simulink library "loco_native_lib"  (R2024b)
settings: Solver=VariableStepAuto  StartTime=0.0  StopTime=10.0  RelTol=1e-3
undefined symbols (not defined in the file): P, PN
libraries: fl_lib x96, nesl_utility x44, $bdroot x21, simulink x2, sdl_lib x1, batteryecm_lib x1
(part 2 of 2)

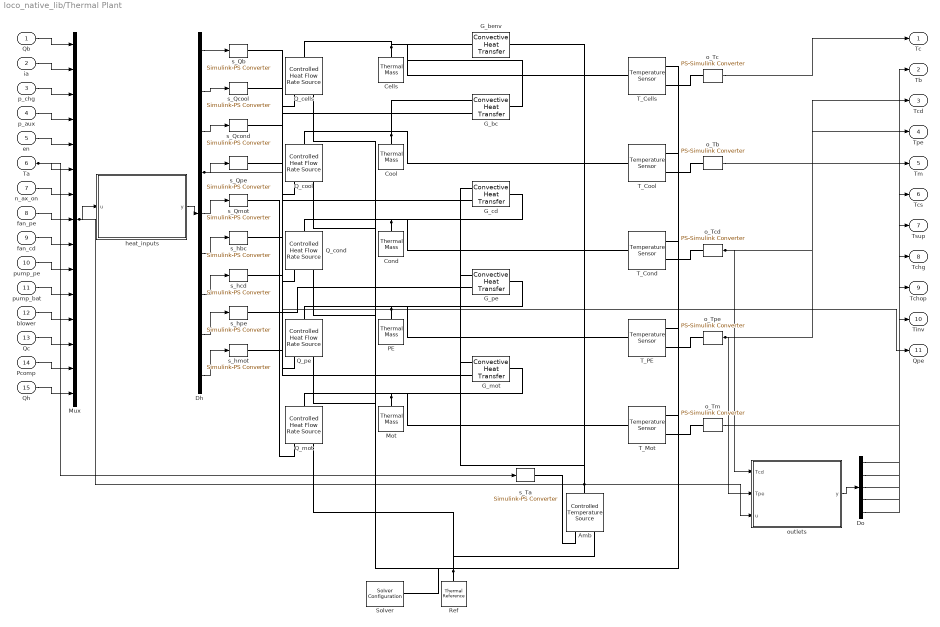
== system loco_native_lib/Thermal Plant ==
  Qb : Inport
  ia : Inport  Port=2
  p_chg : Inport  Port=3
  p_aux : Inport  Port=4
  en : Inport  Port=5
  Ta : Inport  Port=6
  n_ax_on : Inport  Port=7
  fan_pe : Inport  Port=8
  fan_cd : Inport  Port=9
  pump_pe : Inport  Port=10
  pump_bat : Inport  Port=11
  blower : Inport  Port=12
  Qc : Inport  Port=13
  Pcomp : Inport  Port=14
  Qh : Inport  Port=15
  Amb : fl_lib/Thermal/Thermal Sources/Controlled Temperature Source
  Cells : fl_lib/Thermal/Thermal Elements/Thermal Mass  mass_type=foundation.enum.constant_variable.constant  mass=TH.C_bat kg  sp_heat=1 J/(K*kg)  mass_min=1e-6 kg  num_ports=foundation.enum.numPorts2.one  m_specify=off  m_priority=High  m=1 kg  m_nominal_specify=off  m_nominal_value=1  m_nominal_unit=kg  T_specify=on  T_priority=High  T=TH.T0_bat K  T_nominal_specify=off  T_nominal_value=1  T_nominal_unit=K  Q_specify=off  Q_priority=None  Q=0 W  Q_nominal_specify=off  Q_nominal_value=1  Q_nominal_unit=W
  Cond : fl_lib/Thermal/Thermal Elements/Thermal Mass  mass_type=foundation.enum.constant_variable.constant  mass=TH.C_cd kg  sp_heat=1 J/(K*kg)  mass_min=1e-6 kg  num_ports=foundation.enum.numPorts2.one  m_specify=off  m_priority=High  m=1 kg  m_nominal_specify=off  m_nominal_value=1  m_nominal_unit=kg  T_specify=on  T_priority=High  T=TH.T_amb K  T_nominal_specify=off  T_nominal_value=1  T_nominal_unit=K  Q_specify=off  Q_priority=None  Q=0 W  Q_nominal_specify=off  Q_nominal_value=1  Q_nominal_unit=W
  Cool : fl_lib/Thermal/Thermal Elements/Thermal Mass  mass_type=foundation.enum.constant_variable.constant  mass=TH.C_bc kg  sp_heat=1 J/(K*kg)  mass_min=1e-6 kg  num_ports=foundation.enum.numPorts2.one  m_specify=off  m_priority=High  m=1 kg  m_nominal_specify=off  m_nominal_value=1  m_nominal_unit=kg  T_specify=on  T_priority=High  T=TH.T0_bat K  T_nominal_specify=off  T_nominal_value=1  T_nominal_unit=K  Q_specify=off  Q_priority=None  Q=0 W  Q_nominal_specify=off  Q_nominal_value=1  Q_nominal_unit=W
  Dh : Demux  Outputs=9
  Do : Demux  Outputs=5
  G_bc : fl_lib/Thermal/Thermal Elements/Convective Heat Transfer  thermal_type=foundation.enum.constant_variable.variable  area=1 m^2  heat_tr_coeff=20 W/(K*m^2)  min_heat_tr_coeff=1e-3 W/(K*m^2)  T_specify=off  T_priority=None  T=0 K  T_nominal_specify=off  T_nominal_value=1  T_nominal_unit=K  Q_specify=off  Q_priority=None  Q=0 W  Q_nominal_specify=off  Q_nominal_value=1  Q_nominal_unit=W
      settings: InternalSimscapePortConfiguration="{\"Bottom\":[],\"Left\":[{\"id\":\"A\",\"label\":\"A\",\"type\":\"foundation.thermal.thermal\"},{\"id\":\"var_heat_tr_coeff\",\"label\":\"K\",\"type\":\"input\"}],\"Right\":[{\"id\":\"B\",\"label\":\"B\",\"type\":\"foundation.thermal.thermal\"}],\"Top\":[]}"
  G_benv : fl_lib/Thermal/Thermal Elements/Convective Heat Transfer  thermal_type=foundation.enum.constant_variable.constant  area=1 m^2  heat_tr_coeff=TH.UA_benv W/(K*m^2)  min_heat_tr_coeff=1e-3 W/(K*m^2)  T_specify=off  T_priority=None  T=0 K  T_nominal_specify=off  T_nominal_value=1  T_nominal_unit=K  Q_specify=off  Q_priority=None  Q=0 W  Q_nominal_specify=off  Q_nominal_value=1  Q_nominal_unit=W
  G_cd : fl_lib/Thermal/Thermal Elements/Convective Heat Transfer  thermal_type=foundation.enum.constant_variable.variable  area=1 m^2  heat_tr_coeff=20 W/(K*m^2)  min_heat_tr_coeff=1e-3 W/(K*m^2)  T_specify=off  T_priority=None  T=0 K  T_nominal_specify=off  T_nominal_value=1  T_nominal_unit=K  Q_specify=off  Q_priority=None  Q=0 W  Q_nominal_specify=off  Q_nominal_value=1  Q_nominal_unit=W
      settings: InternalSimscapePortConfiguration="{\"Bottom\":[],\"Left\":[{\"id\":\"A\",\"label\":\"A\",\"type\":\"foundation.thermal.thermal\"},{\"id\":\"var_heat_tr_coeff\",\"label\":\"K\",\"type\":\"input\"}],\"Right\":[{\"id\":\"B\",\"label\":\"B\",\"type\":\"foundation.thermal.thermal\"}],\"Top\":[]}"
  G_mot : fl_lib/Thermal/Thermal Elements/Convective Heat Transfer  thermal_type=foundation.enum.constant_variable.variable  area=1 m^2  heat_tr_coeff=20 W/(K*m^2)  min_heat_tr_coeff=1e-3 W/(K*m^2)  T_specify=off  T_priority=None  T=0 K  T_nominal_specify=off  T_nominal_value=1  T_nominal_unit=K  Q_specify=off  Q_priority=None  Q=0 W  Q_nominal_specify=off  Q_nominal_value=1  Q_nominal_unit=W
      settings: InternalSimscapePortConfiguration="{\"Bottom\":[],\"Left\":[{\"id\":\"A\",\"label\":\"A\",\"type\":\"foundation.thermal.thermal\"},{\"id\":\"var_heat_tr_coeff\",\"label\":\"K\",\"type\":\"input\"}],\"Right\":[{\"id\":\"B\",\"label\":\"B\",\"type\":\"foundation.thermal.thermal\"}],\"Top\":[]}"
  G_pe : fl_lib/Thermal/Thermal Elements/Convective Heat Transfer  thermal_type=foundation.enum.constant_variable.variable  area=1 m^2  heat_tr_coeff=20 W/(K*m^2)  min_heat_tr_coeff=1e-3 W/(K*m^2)  T_specify=off  T_priority=None  T=0 K  T_nominal_specify=off  T_nominal_value=1  T_nominal_unit=K  Q_specify=off  Q_priority=None  Q=0 W  Q_nominal_specify=off  Q_nominal_value=1  Q_nominal_unit=W
      settings: InternalSimscapePortConfiguration="{\"Bottom\":[],\"Left\":[{\"id\":\"A\",\"label\":\"A\",\"type\":\"foundation.thermal.thermal\"},{\"id\":\"var_heat_tr_coeff\",\"label\":\"K\",\"type\":\"input\"}],\"Right\":[{\"id\":\"B\",\"label\":\"B\",\"type\":\"foundation.thermal.thermal\"}],\"Top\":[]}"
  Mot : fl_lib/Thermal/Thermal Elements/Thermal Mass  mass_type=foundation.enum.constant_variable.constant  mass=TH.C_mot kg  sp_heat=1 J/(K*kg)  mass_min=1e-6 kg  num_ports=foundation.enum.numPorts2.one  m_specify=off  m_priority=High  m=1 kg  m_nominal_specify=off  m_nominal_value=1  m_nominal_unit=kg  T_specify=on  T_priority=High  T=TH.T_amb K  T_nominal_specify=off  T_nominal_value=1  T_nominal_unit=K  Q_specify=off  Q_priority=None  Q=0 W  Q_nominal_specify=off  Q_nominal_value=1  Q_nominal_unit=W
  Mux : Mux  Inputs=15
  PE : fl_lib/Thermal/Thermal Elements/Thermal Mass  mass_type=foundation.enum.constant_variable.constant  mass=TH.C_pe kg  sp_heat=1 J/(K*kg)  mass_min=1e-6 kg  num_ports=foundation.enum.numPorts2.one  m_specify=off  m_priority=High  m=1 kg  m_nominal_specify=off  m_nominal_value=1  m_nominal_unit=kg  T_specify=on  T_priority=High  T=TH.T_amb K  T_nominal_specify=off  T_nominal_value=1  T_nominal_unit=K  Q_specify=off  Q_priority=None  Q=0 W  Q_nominal_specify=off  Q_nominal_value=1  Q_nominal_unit=W
  Q_cells : fl_lib/Thermal/Thermal Sources/Controlled Heat Flow Rate Source
  Q_cond : fl_lib/Thermal/Thermal Sources/Controlled Heat Flow Rate Source
  Q_cool : fl_lib/Thermal/Thermal Sources/Controlled Heat Flow Rate Source
  Q_mot : fl_lib/Thermal/Thermal Sources/Controlled Heat Flow Rate Source
  Q_pe : fl_lib/Thermal/Thermal Sources/Controlled Heat Flow Rate Source
  Ref : fl_lib/Thermal/Thermal Elements/Thermal Reference
  Solver : nesl_utility/Solver Configuration  PhysicalDomain=network_engine_domain  SubClassName=solver  LeftPortType=input  RightPortType=generic  Tones=[]  Harmonics=[]  SimulateNoise=off  Profile=off  UseLocalSampling=off  EnableSwitchedLinearOptims=on  FrequencyDomain=off  UseCCode=off  RelTol=0.001  AbsTol=0.001  MinStep=1e-09  ToWorkspace=off  RevertToSquareIcSolve=off  NumHomotopyIterations=100  PhasorMode=off  PhasorModeNumHarmonics=1  ConsistencySolver=NEWTON_XTOL_AFTER_FTOL  IndexReductionMethod=DerivativeReplacement  DoDC=off  ResidualTolerance=1e-09  ConsistencyTolSource=GLOBAL  ConsistencyAbsTol=0.001  ConsistencyRelTol=0.001  ConsistencyTolFactor=0.001  UseLocalSolver=off  LocalSolverChoice=NE_BACKWARD_EULER_ADVANCER  ResolveIndetEquations=on  FunctionEvalNumThread=1  LocalSolverSampleTime=0.001  DoFixedCost=off  MaxNonlinIter=3  MaxModeIter=2  ComputeImpulses=off  ImpulseIterations=2  LinearAlgebra=auto  LinearAlgebraNumThread=0  EquationFormulation=NE_TIME_EF  DelaysMemoryBudget=1024  AutomaticFiltering=on  FilteringTimeConstant=0.001  PartitionStorageMethod=AS_NEEDED  PartitionMemoryBudget=1024  PartitionMethod=ROBUST  MultibodyUseLocalSolver=off  MultibodyLocalSolverChoice=ODE1  MultibodyLocalSolverSampleTime=0.001
  T_Cells : fl_lib/Thermal/Thermal Sensors/Temperature Sensor  temperature_measure=foundation.enum.MeasurementReference.difference
  T_Cond : fl_lib/Thermal/Thermal Sensors/Temperature Sensor  temperature_measure=foundation.enum.MeasurementReference.difference
  T_Cool : fl_lib/Thermal/Thermal Sensors/Temperature Sensor  temperature_measure=foundation.enum.MeasurementReference.difference
  T_Mot : fl_lib/Thermal/Thermal Sensors/Temperature Sensor  temperature_measure=foundation.enum.MeasurementReference.difference
  T_PE : fl_lib/Thermal/Thermal Sensors/Temperature Sensor  temperature_measure=foundation.enum.MeasurementReference.difference
  heat_inputs : MATLAB Function  TreatAsAtomicUnit=on
  o_Tb : nesl_utility/PS-Simulink Converter  PhysicalDomain=network_engine_domain  SubClassName=ps_output  LeftPortType=input  RightPortType=output  PseudoPeriodic=off  Frequencies=[]  VectorFormat=inherit  Unit=K  AffineConversion=off
  o_Tc : nesl_utility/PS-Simulink Converter  PhysicalDomain=network_engine_domain  SubClassName=ps_output  LeftPortType=input  RightPortType=output  PseudoPeriodic=off  Frequencies=[]  VectorFormat=inherit  Unit=K  AffineConversion=off
  o_Tcd : nesl_utility/PS-Simulink Converter  PhysicalDomain=network_engine_domain  SubClassName=ps_output  LeftPortType=input  RightPortType=output  PseudoPeriodic=off  Frequencies=[]  VectorFormat=inherit  Unit=K  AffineConversion=off
  o_Tm : nesl_utility/PS-Simulink Converter  PhysicalDomain=network_engine_domain  SubClassName=ps_output  LeftPortType=input  RightPortType=output  PseudoPeriodic=off  Frequencies=[]  VectorFormat=inherit  Unit=K  AffineConversion=off
  o_Tpe : nesl_utility/PS-Simulink Converter  PhysicalDomain=network_engine_domain  SubClassName=ps_output  LeftPortType=input  RightPortType=output  PseudoPeriodic=off  Frequencies=[]  VectorFormat=inherit  Unit=K  AffineConversion=off
  outlets : MATLAB Function  TreatAsAtomicUnit=on
  s_Qb : nesl_utility/Simulink-PS Converter  PhysicalDomain=network_engine_domain  SubClassName=ps_input  LeftPortType=input  RightPortType=output  PseudoPeriodic=off  Frequencies=[]  NoiseDistribution=none  NoiseParameters=[]  Unit=W  AffineConversion=off  FilteringAndDerivatives=provide  SimscapeFilterOrder=1  InputFilterTimeConstant=0.001  UdotUserProvided=0
  s_Qcond : nesl_utility/Simulink-PS Converter  PhysicalDomain=network_engine_domain  SubClassName=ps_input  LeftPortType=input  RightPortType=output  PseudoPeriodic=off  Frequencies=[]  NoiseDistribution=none  NoiseParameters=[]  Unit=W  AffineConversion=off  FilteringAndDerivatives=provide  SimscapeFilterOrder=1  InputFilterTimeConstant=0.001  UdotUserProvided=0
  s_Qcool : nesl_utility/Simulink-PS Converter  PhysicalDomain=network_engine_domain  SubClassName=ps_input  LeftPortType=input  RightPortType=output  PseudoPeriodic=off  Frequencies=[]  NoiseDistribution=none  NoiseParameters=[]  Unit=W  AffineConversion=off  FilteringAndDerivatives=provide  SimscapeFilterOrder=1  InputFilterTimeConstant=0.001  UdotUserProvided=0
  s_Qmot : nesl_utility/Simulink-PS Converter  PhysicalDomain=network_engine_domain  SubClassName=ps_input  LeftPortType=input  RightPortType=output  PseudoPeriodic=off  Frequencies=[]  NoiseDistribution=none  NoiseParameters=[]  Unit=W  AffineConversion=off  FilteringAndDerivatives=provide  SimscapeFilterOrder=1  InputFilterTimeConstant=0.001  UdotUserProvided=0
  s_Qpe : nesl_utility/Simulink-PS Converter  PhysicalDomain=network_engine_domain  SubClassName=ps_input  LeftPortType=input  RightPortType=output  PseudoPeriodic=off  Frequencies=[]  NoiseDistribution=none  NoiseParameters=[]  Unit=W  AffineConversion=off  FilteringAndDerivatives=provide  SimscapeFilterOrder=1  InputFilterTimeConstant=0.001  UdotUserProvided=0
  s_Ta : nesl_utility/Simulink-PS Converter  PhysicalDomain=network_engine_domain  SubClassName=ps_input  LeftPortType=input  RightPortType=output  PseudoPeriodic=off  Frequencies=[]  NoiseDistribution=none  NoiseParameters=[]  Unit=K  AffineConversion=off  FilteringAndDerivatives=provide  SimscapeFilterOrder=1  InputFilterTimeConstant=0.001  UdotUserProvided=0
  s_hbc : nesl_utility/Simulink-PS Converter  PhysicalDomain=network_engine_domain  SubClassName=ps_input  LeftPortType=input  RightPortType=output  PseudoPeriodic=off  Frequencies=[]  NoiseDistribution=none  NoiseParameters=[]  Unit=W/(m^2*K)  AffineConversion=off  FilteringAndDerivatives=provide  SimscapeFilterOrder=1  InputFilterTimeConstant=0.001  UdotUserProvided=0
  s_hcd : nesl_utility/Simulink-PS Converter  PhysicalDomain=network_engine_domain  SubClassName=ps_input  LeftPortType=input  RightPortType=output  PseudoPeriodic=off  Frequencies=[]  NoiseDistribution=none  NoiseParameters=[]  Unit=W/(m^2*K)  AffineConversion=off  FilteringAndDerivatives=provide  SimscapeFilterOrder=1  InputFilterTimeConstant=0.001  UdotUserProvided=0
  s_hmot : nesl_utility/Simulink-PS Converter  PhysicalDomain=network_engine_domain  SubClassName=ps_input  LeftPortType=input  RightPortType=output  PseudoPeriodic=off  Frequencies=[]  NoiseDistribution=none  NoiseParameters=[]  Unit=W/(m^2*K)  AffineConversion=off  FilteringAndDerivatives=provide  SimscapeFilterOrder=1  InputFilterTimeConstant=0.001  UdotUserProvided=0
  s_hpe : nesl_utility/Simulink-PS Converter  PhysicalDomain=network_engine_domain  SubClassName=ps_input  LeftPortType=input  RightPortType=output  PseudoPeriodic=off  Frequencies=[]  NoiseDistribution=none  NoiseParameters=[]  Unit=W/(m^2*K)  AffineConversion=off  FilteringAndDerivatives=provide  SimscapeFilterOrder=1  InputFilterTimeConstant=0.001  UdotUserProvided=0
  Tc : Outport
  Tb : Outport  Port=2
  Tcd : Outport  Port=3
  Tpe : Outport  Port=4
  Tm : Outport  Port=5
  Tcs : Outport  Port=6
  Tsup : Outport  Port=7
  Tchg : Outport  Port=8
  Tchop : Outport  Port=9
  Tinv : Outport  Port=10
  Qpe : Outport  Port=11
  wires:
  Qb/1 -> Mux/1
  ia/1 -> Mux/2
  p_chg/1 -> Mux/3
  p_aux/1 -> Mux/4
  en/1 -> Mux/5
  Ta/1 -> Mux/6, s_Ta/1
  n_ax_on/1 -> Mux/7
  fan_pe/1 -> Mux/8
  fan_cd/1 -> Mux/9
  pump_pe/1 -> Mux/10
  pump_bat/1 -> Mux/11
  blower/1 -> Mux/12
  Qc/1 -> Mux/13
  Pcomp/1 -> Mux/14
  Qh/1 -> Mux/15
  Mux/1 -> heat_inputs/1(u), outlets/3(u)
  heat_inputs/1(y) -> Dh/1
  Dh/1 -> s_Qb/1
  Dh/2 -> s_Qcool/1
  Dh/3 -> s_Qcond/1
  Dh/4 -> s_Qpe/1, Qpe/1
  Dh/5 -> s_Qmot/1
  Dh/6 -> s_hbc/1
  Dh/7 -> s_hcd/1
  Dh/8 -> s_hpe/1
  Dh/9 -> s_hmot/1
  o_Tcd/1 -> outlets/1(Tcd), Tcd/1
  o_Tpe/1 -> outlets/2(Tpe), Tpe/1
  outlets/1(y) -> Do/1
  o_Tc/1 -> Tc/1
  o_Tb/1 -> Tb/1
  o_Tm/1 -> Tm/1
  Do/1 -> Tcs/1
  Do/2 -> Tsup/1
  Do/3 -> Tchg/1
  Do/4 -> Tchop/1
  Do/5 -> Tinv/1
  connections:
  Solver/RConn1 -- Amb/RConn2 -- Q_cells/RConn2 -- T_Cells/RConn1 -- Q_cool/RConn2 -- T_Cool/RConn1 -- Q_cond/RConn2 -- T_Cond/RConn1 -- Q_pe/RConn2 -- T_PE/RConn1 -- Q_mot/RConn2 -- Ref/LConn1 -- T_Mot/RConn1
  s_Ta/RConn1 -- Amb/RConn1
  s_Qb/RConn1 -- Q_cells/RConn1
  Q_cells/LConn1 -- T_Cells/LConn1 -- G_benv/LConn1 -- Cells/LConn1 -- G_bc/RConn1
  T_Cells/RConn2 -- o_Tc/LConn1
  s_Qcool/RConn1 -- Q_cool/RConn1
  Q_cool/LConn1 -- T_Cool/LConn1 -- Cool/LConn1 -- G_bc/LConn1
  T_Cool/RConn2 -- o_Tb/LConn1
  s_Qcond/RConn1 -- Q_cond/RConn1
  Q_cond/LConn1 -- T_Cond/LConn1 -- Cond/LConn1 -- G_cd/RConn1
  T_Cond/RConn2 -- o_Tcd/LConn1
  s_Qpe/RConn1 -- Q_pe/RConn1
  Q_pe/LConn1 -- T_PE/LConn1 -- PE/LConn1 -- G_pe/RConn1
  T_PE/RConn2 -- o_Tpe/LConn1
  s_Qmot/RConn1 -- Q_mot/RConn1
  Q_mot/LConn1 -- T_Mot/LConn1 -- Mot/LConn1 -- G_mot/RConn1
  T_Mot/RConn2 -- o_Tm/LConn1
  G_benv/RConn1 -- G_cd/LConn1 -- G_pe/LConn1 -- Amb/LConn1 -- G_mot/LConn1
  s_hbc/RConn1 -- G_bc/LConn2
  s_hcd/RConn1 -- G_cd/LConn2
  s_hpe/RConn1 -- G_pe/LConn2
  s_hmot/RConn1 -- G_mot/LConn2

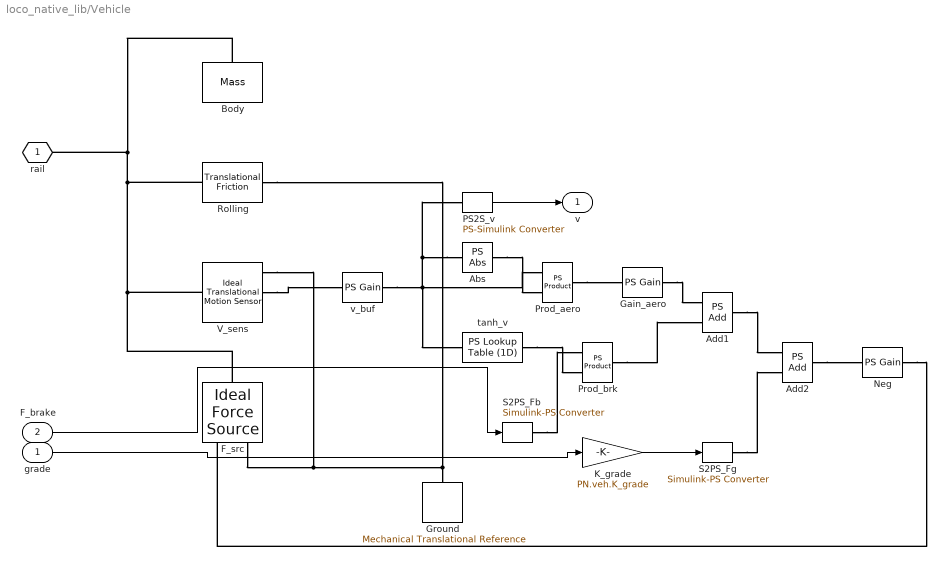
== system loco_native_lib/Vehicle ==
  grade : Inport
  F_brake : Inport  Port=2
  Abs : fl_lib/Physical Signals/Nonlinear Operators/PS Abs
      settings: InternalSimscapePortConfiguration="{\"Bottom\":[],\"Left\":[{\"id\":\"I\",\"label\":\"\",\"type\":\"input\"}],\"Right\":[{\"id\":\"O\",\"label\":\"\",\"type\":\"output\"}],\"Top\":[]}"
  Add1 : fl_lib/Physical Signals/Functions/PS Add
  Add2 : fl_lib/Physical Signals/Functions/PS Add
  Body : fl_lib/Mechanical/Translational Elements/Mass  mass=PN.veh.m_eff kg  num_ports=foundation.enum.numPorts2.one  v_specify=on  v_priority=High  v=PN.veh.v0 m/s  v_nominal_specify=off  v_nominal_value=1  v_nominal_unit=m/s  f_specify=off  f_priority=None  f=0 N  f_nominal_specify=off  f_nominal_value=1  f_nominal_unit=N
  F_src : fl_lib/Mechanical/Mechanical Sources/Ideal Force Source
  Gain_aero : fl_lib/Physical Signals/Functions/PS Gain  gain=PN.veh.k_aero N*s^2/m^2
  Ground : fl_lib/Mechanical/Translational Elements/Mechanical Translational Reference
  K_grade : Gain  Gain=PN.veh.K_grade
  Neg : fl_lib/Physical Signals/Functions/PS Gain  gain=-1
  PS2S_v : nesl_utility/PS-Simulink Converter  PhysicalDomain=network_engine_domain  SubClassName=ps_output  LeftPortType=input  RightPortType=output  PseudoPeriodic=off  Frequencies=[]  VectorFormat=inherit  Unit=m/s  AffineConversion=off
  Prod_aero : fl_lib/Physical Signals/Functions/PS Product
  Prod_brk : fl_lib/Physical Signals/Functions/PS Product
  Rolling : fl_lib/Mechanical/Translational Elements/Translational Friction  brkwy_frc=PN.veh.F_roll N  brkwy_vel=1 m/s  Col_frc=PN.veh.F_roll N  visc_coef=0 N*s/m  v_specify=off  v_priority=None  v=0 m/s  v_nominal_specify=off  v_nominal_value=1  v_nominal_unit=m/s  f_specify=off  f_priority=None  f=0 N  f_nominal_specify=off  f_nominal_value=1  f_nominal_unit=N
      settings: InternalSimscapePortConfiguration="{\"Bottom\":[],\"Left\":[{\"id\":\"R\",\"label\":\"R\",\"type\":\"foundation.mechanical.translational.translational\"}],\"Right\":[{\"id\":\"C\",\"label\":\"C\",\"type\":\"foundation.mechanical.translational.translational\"}],\"Top\":[]}"
  S2PS_Fb : nesl_utility/Simulink-PS Converter  PhysicalDomain=network_engine_domain  SubClassName=ps_input  LeftPortType=input  RightPortType=output  PseudoPeriodic=off  Frequencies=[]  NoiseDistribution=none  NoiseParameters=[]  Unit=N  AffineConversion=off  FilteringAndDerivatives=provide  SimscapeFilterOrder=1  InputFilterTimeConstant=0.001  UdotUserProvided=0
  S2PS_Fg : nesl_utility/Simulink-PS Converter  PhysicalDomain=network_engine_domain  SubClassName=ps_input  LeftPortType=input  RightPortType=output  PseudoPeriodic=off  Frequencies=[]  NoiseDistribution=none  NoiseParameters=[]  Unit=N  AffineConversion=off  FilteringAndDerivatives=provide  SimscapeFilterOrder=1  InputFilterTimeConstant=0.001  UdotUserProvided=0
  V_sens : fl_lib/Mechanical/Mechanical Sensors/Ideal Translational Motion Sensor  reference=foundation.enum.MeasurementReference.difference  acceleration_port=false  velocity_port=true  position_port=true  offset=0 m
  tanh_v : fl_lib/Physical Signals/Lookup Tables/PS Lookup Table (1D)  x=PN.veh.tanh_x m/s  f=PN.veh.tanh_f  interp_method=simscape.enum.interpolation.linear  extrap_method=simscape.enum.extrapolation.linear
  v_buf : fl_lib/Physical Signals/Functions/PS Gain  gain=1
  rail : PMIOPort  Side=Left
  v : Outport
  wires:
  grade/1 -> K_grade/1
  K_grade/1 -> S2PS_Fg/1
  F_brake/1 -> S2PS_Fb/1
  PS2S_v/1 -> v/1
  connections:
  Abs/LConn1 -- v_buf/RConn1 -- Prod_aero/LConn1 -- tanh_v/LConn1 -- PS2S_v/LConn1
  Abs/RConn1 -- Prod_aero/LConn2
  Prod_aero/RConn1 -- Gain_aero/LConn1
  S2PS_Fb/RConn1 -- Prod_brk/LConn1
  tanh_v/RConn1 -- Prod_brk/LConn2
  Gain_aero/RConn1 -- Add1/LConn1
  Prod_brk/RConn1 -- Add1/LConn2
  Add1/RConn1 -- Add2/LConn1
  S2PS_Fg/RConn1 -- Add2/LConn2
  Add2/RConn1 -- Neg/LConn1
  Body/LConn1 -- F_src/LConn1 -- V_sens/LConn1 -- Rolling/LConn1 -- rail/RConn1
  Rolling/RConn1 -- F_src/RConn2 -- V_sens/RConn1 -- Ground/LConn1
  V_sens/RConn2 -- v_buf/LConn1
  Neg/RConn1 -- F_src/RConn1

== matlab function loco_native_lib/LCC/lcc ==
  data: u input size=[9 1]; y output; L parameter
function y = lcc(u, L)
persistent xi
if isempty(xi), xi = 0; end
v_ref = u(1); v = u(2); Vbat = u(3); k_dis = u(4); k_chg = u(5);
m_trail = u(6); trac = u(7); n_ax_on = u(8); n_str = u(9);
mt = max(m_trail, 0);
m_tot = L.m_loco + mt;
m_eff = L.k_rot_loco*L.m_loco + L.k_rot_trail*mt;
Kp = 2*L.zeta*L.wn*m_eff;
Ki = L.wn^2*m_eff;
nax = min(max(n_ax_on, 0), L.N_ax);
fstr = min(max(n_str, 0), L.N_str_nom)/L.N_str_nom;
TE_adh = L.mu_adh*L.m_loco*L.g*nax/L.N_ax;
e = v_ref - v;
TE_raw = Kp*e + xi;
vabs = max(abs(v), L.v_floor);
P_dis = trac*min(L.P_trac_max*nax/L.N_ax, L.I_dis_max*fstr*k_dis*Vbat*L.eta_drv);
P_reg = min(L.P_trac_max*nax/L.N_ax, L.I_chg_max*fstr*k_chg*Vbat/L.eta_drv);
TE_mot_lim = min(TE_adh, P_dis/vabs);
TE_reg_lim = min(TE_adh, P_reg/vabs)*min(abs(v)/L.v_blend, 1);
TE_cmd = min(max(TE_raw, -TE_adh), TE_mot_lim);
TE_el = max(TE_cmd, -TE_reg_lim);
F_park = L.mu_park*m_tot*L.g;
if v_ref < 0.01
    F_hold = F_park;
    dxi = -xi/1;
else
    F_hold = F_park*min(max(-v/L.v_rb, 0), 1);
    dxi = Ki*e + (TE_cmd - TE_raw)/L.T_aw;
end
xi = xi + L.Ts*dxi;
TE_each = TE_el/max(nax, 1);
y = [TE_each; TE_each*min(max(nax - 3, 0), 1); TE_el - TE_cmd + F_hold];
end

== matlab function loco_native_lib/Chopper FW/fw ==
  data: TE_ref input size=[1 1]; Va output; i_a input size=[1 1]; v input size=[1 1]; Vdc input size=[1 1]; A parameter
function Va = fw(TE_ref, i_a, v, Vdc, A)
wm = A.G*v/A.r_w;
kphi = A.Kphi_sat*(1 - exp(-max(abs(i_a), A.If_min)/A.I0));
E = kphi*wm;
Vmax = min(A.D_max*max(Vdc, 0), A.V_mot_max);
Tm_lim = A.P_ax_max/max(abs(wm), A.w_floor);
Tm_ref = min(max(TE_ref*A.r_w/A.G, -Tm_lim), Tm_lim);
Iref = sign(Tm_ref)*interp1(A.T_tab, A.I_tab, min(abs(Tm_ref), A.T_tab(end)));
Iref = min(max(Iref, -A.I_max), A.I_max);
Va = min(max(E + A.R_m*i_a + A.Kp_i*(Iref - i_a), 0), Vmax);
end

== matlab function loco_native_lib/Charger FW/chg ==
  data: u input size=[5 1]; i output; P_max parameter; I_max parameter; I_bms parameter; soc_max parameter; soc_band parameter; V_floor parameter; N_str_nom parameter
function i = chg(u, P_max, I_max, I_bms, soc_max, soc_band, V_floor, N_str_nom)
P = u(1); k = u(2); soc = u(3); n_str = u(4); V = u(5);
Ilim = min(I_max, I_bms*k*n_str/N_str_nom);
Ip = min(max(P, 0), P_max)/max(V, V_floor);
taper = min(max((soc_max - soc)/soc_band, 0), 1);
i = min(Ip, Ilim)*taper;
end

== matlab function loco_native_lib/Thermal Plant/heat_inputs ==
  data: u input size=[15 1]; y output; TH parameter; f_ram parameter
function y = heat_inputs(u, TH, f_ram)
Qb = u(1); ia = u(2); p_chg = u(3); p_aux = u(4); en = u(5);
n_ax = u(7); fan_pe = u(8); fan_cd = u(9); pump_pe = u(10); pump_bat = u(11);
blower = u(12); Qc = u(13); Pcomp = u(14); Qh = u(15);
Qchop = n_ax*(TH.a_loss*abs(ia) + TH.b_loss*ia^2);
Qchg = max(p_chg, 0)*(1/TH.eta_chg - 1);
Qpe = Qchop + Qchg + TH.k_aux_pe*p_aux + TH.Q_pe_idle*en;
h_bc = TH.UA_bc*(0.2 + 0.8*pump_bat);
h_cd = TH.UA_cd*(f_ram + (1 - f_ram)*fan_cd);
h_pe = TH.UA_pe*(f_ram + (1 - f_ram)*fan_pe)*min(1, 0.2 + 0.8*pump_pe);
h_mot = TH.UA_mot*(0.15 + 0.85*blower);
y = [Qb; Qh - Qc; Qc + Pcomp; Qpe; TH.R_m*ia^2; h_bc; h_cd; h_pe; h_mot];
end

== matlab function loco_native_lib/Thermal Plant/outlets ==
  data: Tcd input size=[1 1]; Tpe input size=[1 1]; u input size=[15 1]; y output; TH parameter; f_ram parameter
function y = outlets(Tcd, Tpe, u, TH, f_ram)
ia = u(2); p_chg = u(3); p_aux = u(4); Ta = u(6);
fan_pe = u(8); fan_cd = u(9); pump_pe = u(10);
Qrad_cd = TH.UA_cd*(f_ram + (1 - f_ram)*fan_cd)*(Tcd - Ta);
Tcs = Tcd - Qrad_cd/TH.mcp_cd;
fq = max(pump_pe, 0.05);
Qrad_pe = TH.UA_pe*(f_ram + (1 - f_ram)*fan_pe)*min(1, 0.2 + 0.8*pump_pe)*(Tpe - Ta);
Tsup = Tpe - Qrad_pe/(TH.mcp_pe*fq);
Qchg = max(p_chg, 0)*(1/TH.eta_chg - 1);
Tchg = Tsup + Qchg/(TH.mcp_chg*fq);
Tchop = Tsup + (TH.a_loss*abs(ia) + TH.b_loss*ia^2)/(TH.mcp_chop*fq);
Tinv = Tsup + TH.k_inv*p_aux/(TH.mcp_inv*fq);
y = [Tcs; Tsup; Tchg; Tchop; Tinv];
end

== matlab function loco_native_lib/TMS Controller/tms ==
  data: u input size=[9 1]; y output; TH parameter; Ts parameter
function y = tms(u, TH, Ts)
persistent mc mh
if isempty(mc), mc = 0; mh = 0; end
Tc = u(1); Tcs = u(2); Tpe = u(3); dT_s = u(4); tms_en = u(5);
n_mtm = u(6); en = u(7); fan_cd = u(8); fan_pe = u(9);
Tsens = Tc + dT_s;
f1 = min(max(1 - TH.k_cap*(Tcs - TH.T_cs_ref), 0), 1.2);
f2 = min(max((TH.T_cs_cut - Tcs)/TH.dT_cut, 0), 1);
Qc_av = min(max(n_mtm, 0), TH.N_mtm)*TH.Q_mtm*f1*f2;
Qc = tms_en*mc*min(max(TH.Kp_chill*(Tsens - TH.T_cool_set), 0), Qc_av);
COP = max(TH.COP_min, TH.COP_ref - TH.k_cop*(Tcs - TH.T_cs_ref));
Pcomp = Qc/COP;
Qh = tms_en*mh*TH.Q_heat_max;
f_pe = min(max((Tpe - TH.T_fan_on)/TH.dT_fan, 0.1), 1);
Ptms = Pcomp + Qh + TH.P_pump*tms_en + TH.P_fan_cd*mc*tms_en*fan_cd + TH.P_fan_pe*f_pe*en*fan_pe;
k_hot = min(max((TH.T_hot_L2 - Tsens)/(TH.T_hot_L2 - TH.T_hot_L1), 0), 1);
k_cc = min(max((Tsens - TH.T_cchg_L2)/(TH.T_cchg_L1 - TH.T_cchg_L2), 0), 1);
k_cd = min(max((Tsens - TH.T_cdis_L2)/(TH.T_cdis_L1 - TH.T_cdis_L2), 0), 1);
tc = double(Tsens >= TH.T_cool_on || (mc > 0.5 && Tsens > TH.T_cool_off));
th = double(Tsens <= TH.T_heat_on || (mh > 0.5 && Tsens < TH.T_heat_off));
y = [Qc; Pcomp; Qh; Ptms; k_hot*k_cd; k_hot*k_cc; mc; mh];
mc = mc + Ts/TH.tau_m*(tc - mc);
mh = mh + Ts/TH.tau_m*(th - mh);
end

== matlab function loco_native_lib/Native Plant/plant_inputs ==
  data: speed_ref_mph input; u output; grade_pct input; ambient_C input; trailing_tons input; cmd input; flt input
function u = plant_inputs(speed_ref_mph, grade_pct, ambient_C, trailing_tons, cmd, flt)
u = zeros(18, 1);
u(1) = max(speed_ref_mph, 0);
u(2) = grade_pct;
u(3) = cmd(5);
u(4) = cmd(6);
u(5) = cmd(2);
u(6) = ambient_C + 273.15;
u(7) = max(trailing_tons, 0)*907.185;
u(8) = cmd(3);
u(9:16) = flt(1:8);
u(17) = flt(9)*flt(11);
u(18) = cmd(4);
end

== matlab function loco_native_lib/Native Plant/pack_soc ==
  data: s input; soc output; K input
function soc = pack_soc(s, K)
n = sum(K);
if n > 0
    soc = sum(s(:).*K(:))/n;
else
    soc = mean(s);
end
end
